simulink model "two_RC_model"  (R2024b)
settings: Solver=VariableStepAuto  StartTime=0.0  StopTime=5000  RelTol=1e-3
undefined symbols (not defined in the file or in its folder): sigbuilder_block
settings Model: Creator=Administrator  LastModifiedBy=sk3547969879
settings DebuggingCC: UnconnectedInputMsg=warning  UnconnectedOutputMsg=warning  UnconnectedLineMsg=warning
settings ModelReferenceCC: EnableRefExpFcnMdlSchedulingChecks=on
settings RTWCC: GPUComputeCapability=3.5  DLArmComputeVersion=19.05

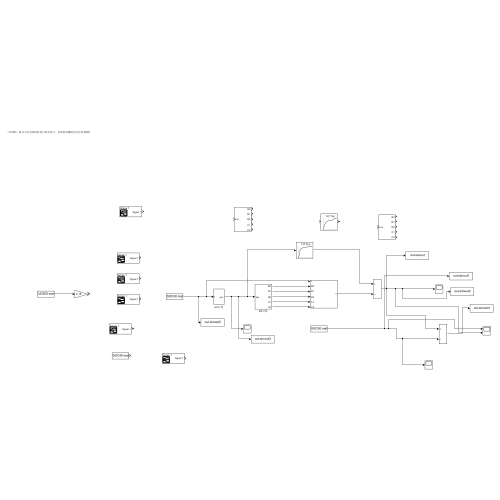
[thumbnail: Simulink's stored preview of the top-level diagram]
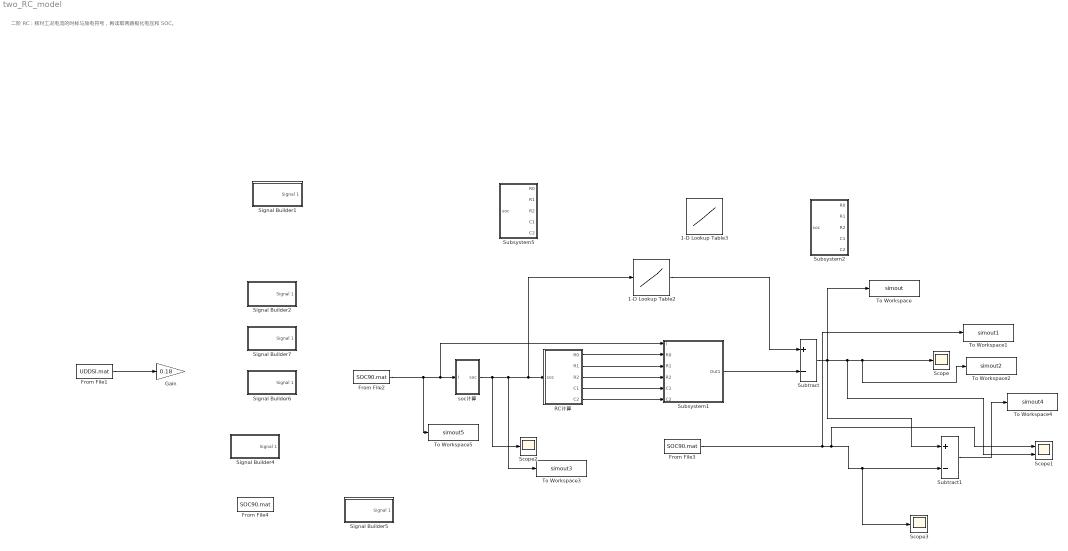
== system two_RC_model ==
  note: 二阶 RC：核对工况电流的时标与放电符号，再读取两路极化电压和 SOC。
  1-D Lookup Table2 : Lookup_n-D  NumberOfTableDimensions=1  BreakpointsForDimension1=[0 0.1 0.2 0.3 0.4 0.5 0.6 0.7 0.8 0.9]  Table=|  InternalRulePriority=Speed  RndMeth=Simplest
      | [2.73200000000000
      | 3.16400000000000
      | 3.21900000000000
      | 3.26100000000000
      | 3.28700000000000
      | 3.28800000000000
      | 3.29100000000000
      | 3.32800000000000
      | 3.32800000000000
      | 3.32900000000000]
  1-D Lookup Table3 : Lookup_n-D  NumberOfTableDimensions=1  BreakpointsForDimension1=[0.1 0.2 0.3 0.4 0.5 0.6 0.7 0.8 0.9]  Table=|  InternalRulePriority=Speed  RndMeth=Simplest
      | [12.8525
      | 13.1367
      | 13.3425
      | 13.3736
      | 13.39
      | 13.4033
      | 13.4506
      | 13.5189
      | 13.5482
      | ]
  From File1 : FromFile  FileName=UDDSI.mat  SampleTime=0
  From File2 : FromFile  FileName=SOC90.mat  SampleTime=0
  From File3 : FromFile  FileName=SOC90.mat  SampleTime=0
  From File4 : FromFile  FileName=SOC90.mat  SampleTime=0
  Gain : Gain  Gain=0.18
  RC计算 : Subsystem
  Scope : Scope
  Scope1 : Scope  NumInputPorts=2
  Scope2 : Scope
  Scope3 : Scope
  Signal Builder1 : Subsystem  Tag=STV Subsys  LoadFcn=sigbuilder_block('load');  StartFcn=sigbuilder_block('start');  StopFcn=sigbuilder_block('stop');  ClipboardFcn=sigbuilder_block('clipboard');  mask(Sigbuilder block){tuvar=[0:10]}
      mask help: Simulink:masks:SigbuilderBlock_MD
      mask init:
      | if ~strcmp(get_param(bdroot(gcbh),'SimulationStatus'),'stopped') tuvar = sigbuilder_block('maskInit'); end
      settings: CopyFcn=sigbuilder_block('copy');  DeleteFcn=sigbuilder_block('delete');  ModelCloseFcn=sigbuilder_block('modelClose');  PreSaveFcn=sigbuilder_block('preSave');  PauseFcn=sigbuilder_block('pause');  ContinueFcn=sigbuilder_block('continue');  NameChangeFcn=sigbuilder_block('namechange');  OpenFcn=sigbuilder_block('open',[437.6 199.2 550.4 400 ]);  CloseFcn=sigbuilder_block('close');
      mask Display: plot(0, 0, 100, 100,[2, 2, 32, 32, 2], [68, 8, 8, 68, 68],[32, 2], [38, 38], [32, 19, 2],[53, 60, 44], [32, 17, 17, 2],[16, 16, 31, 31]);txt = getActiveGroup(gcbh);text(2, 100, txt,'verticalAlignment', 'top');
  Signal Builder2 : Subsystem  Tag=STV Subsys  LoadFcn=sigbuilder_block('load');  StartFcn=sigbuilder_block('start');  StopFcn=sigbuilder_block('stop');  ClipboardFcn=sigbuilder_block('clipboard');  mask(Sigbuilder block){tuvar=[0:10]}
      mask help: Simulink:masks:SigbuilderBlock_MD
      mask init:
      | if ~strcmp(get_param(bdroot(gcbh),'SimulationStatus'),'stopped') tuvar = sigbuilder_block('maskInit'); end
      settings: CopyFcn=sigbuilder_block('copy');  DeleteFcn=sigbuilder_block('delete');  ModelCloseFcn=sigbuilder_block('modelClose');  PreSaveFcn=sigbuilder_block('preSave');  PauseFcn=sigbuilder_block('pause');  ContinueFcn=sigbuilder_block('continue');  NameChangeFcn=sigbuilder_block('namechange');  OpenFcn=sigbuilder_block('open',[437.6 199.2 550.4 400 ]);  CloseFcn=sigbuilder_block('close');
      mask Display: plot(0, 0, 100, 100,[2, 2, 32, 32, 2], [68, 8, 8, 68, 68],[32, 2], [38, 38], [32, 19, 2],[53, 60, 44], [32, 17, 17, 2],[16, 16, 31, 31]);txt = getActiveGroup(gcbh);text(2, 100, txt,'verticalAlignment', 'top');
  Signal Builder4 : Subsystem  Tag=STV Subsys  LoadFcn=sigbuilder_block('load');  StartFcn=sigbuilder_block('start');  StopFcn=sigbuilder_block('stop');  ClipboardFcn=sigbuilder_block('clipboard');  mask(Sigbuilder block){tuvar=[0:10]}
      mask help: Simulink:masks:SigbuilderBlock_MD
      mask init:
      | if ~strcmp(get_param(bdroot(gcbh),'SimulationStatus'),'stopped') tuvar = sigbuilder_block('maskInit'); end
      settings: CopyFcn=sigbuilder_block('copy');  DeleteFcn=sigbuilder_block('delete');  ModelCloseFcn=sigbuilder_block('modelClose');  PreSaveFcn=sigbuilder_block('preSave');  PauseFcn=sigbuilder_block('pause');  ContinueFcn=sigbuilder_block('continue');  NameChangeFcn=sigbuilder_block('namechange');  OpenFcn=sigbuilder_block('open',[6 36 1428 674.25 ]);  CloseFcn=sigbuilder_block('close');
      mask Display: plot(0, 0, 100, 100,[2, 2, 32, 32, 2], [68, 8, 8, 68, 68],[32, 2], [38, 38], [32, 19, 2],[53, 60, 44], [32, 17, 17, 2],[16, 16, 31, 31]);txt = getActiveGroup(gcbh);text(2, 100, txt,'verticalAlignment', 'top');
  Signal Builder5 : Subsystem  Tag=STV Subsys  LoadFcn=sigbuilder_block('load');  StartFcn=sigbuilder_block('start');  StopFcn=sigbuilder_block('stop');  ClipboardFcn=sigbuilder_block('clipboard');  mask(Sigbuilder block){tuvar=[0:10]}
      mask help: Simulink:masks:SigbuilderBlock_MD
      mask init:
      | if ~strcmp(get_param(bdroot(gcbh),'SimulationStatus'),'stopped') tuvar = sigbuilder_block('maskInit'); end
      settings: CopyFcn=sigbuilder_block('copy');  DeleteFcn=sigbuilder_block('delete');  ModelCloseFcn=sigbuilder_block('modelClose');  PreSaveFcn=sigbuilder_block('preSave');  PauseFcn=sigbuilder_block('pause');  ContinueFcn=sigbuilder_block('continue');  NameChangeFcn=sigbuilder_block('namechange');  OpenFcn=sigbuilder_block('open',[437.6 199.2 550.4 400 ]);  CloseFcn=sigbuilder_block('close');
      mask Display: plot(0, 0, 100, 100,[2, 2, 32, 32, 2], [68, 8, 8, 68, 68],[32, 2], [38, 38], [32, 19, 2],[53, 60, 44], [32, 17, 17, 2],[16, 16, 31, 31]);txt = getActiveGroup(gcbh);text(2, 100, txt,'verticalAlignment', 'top');
  Signal Builder6 : Subsystem  Tag=STV Subsys  LoadFcn=sigbuilder_block('load');  StartFcn=sigbuilder_block('start');  StopFcn=sigbuilder_block('stop');  ClipboardFcn=sigbuilder_block('clipboard');  mask(Sigbuilder block){tuvar=[0:10]}
      mask help: Simulink:masks:SigbuilderBlock_MD
      mask init:
      | if ~strcmp(get_param(bdroot(gcbh),'SimulationStatus'),'stopped') tuvar = sigbuilder_block('maskInit'); end
      settings: CopyFcn=sigbuilder_block('copy');  DeleteFcn=sigbuilder_block('delete');  ModelCloseFcn=sigbuilder_block('modelClose');  PreSaveFcn=sigbuilder_block('preSave');  PauseFcn=sigbuilder_block('pause');  ContinueFcn=sigbuilder_block('continue');  NameChangeFcn=sigbuilder_block('namechange');  OpenFcn=sigbuilder_block('open',[437.6 199.2 550.4 400 ]);  CloseFcn=sigbuilder_block('close');
      mask Display: plot(0, 0, 100, 100,[2, 2, 32, 32, 2], [68, 8, 8, 68, 68],[32, 2], [38, 38], [32, 19, 2],[53, 60, 44], [32, 17, 17, 2],[16, 16, 31, 31]);txt = getActiveGroup(gcbh);text(2, 100, txt,'verticalAlignment', 'top');
  Signal Builder7 : Subsystem  Tag=STV Subsys  LoadFcn=sigbuilder_block('load');  StartFcn=sigbuilder_block('start');  StopFcn=sigbuilder_block('stop');  ClipboardFcn=sigbuilder_block('clipboard');  mask(Sigbuilder block){tuvar=[0:10]}
      mask help: Simulink:masks:SigbuilderBlock_MD
      mask init:
      | if ~strcmp(get_param(bdroot(gcbh),'SimulationStatus'),'stopped') tuvar = sigbuilder_block('maskInit'); end
      settings: CopyFcn=sigbuilder_block('copy');  DeleteFcn=sigbuilder_block('delete');  ModelCloseFcn=sigbuilder_block('modelClose');  PreSaveFcn=sigbuilder_block('preSave');  PauseFcn=sigbuilder_block('pause');  ContinueFcn=sigbuilder_block('continue');  NameChangeFcn=sigbuilder_block('namechange');  OpenFcn=sigbuilder_block('open',[4.875 36 1190.25 638.25 ]);  CloseFcn=sigbuilder_block('close');
      mask Display: plot(0, 0, 100, 100,[2, 2, 32, 32, 2], [68, 8, 8, 68, 68],[32, 2], [38, 38], [32, 19, 2],[53, 60, 44], [32, 17, 17, 2],[16, 16, 31, 31]);txt = getActiveGroup(gcbh);text(2, 100, txt,'verticalAlignment', 'top');
  Subsystem1 : Subsystem
  Subsystem2 : Subsystem
  Subsystem5 : Subsystem
  Subtract : Sum  Inputs=+-
  Subtract1 : Sum  Inputs=+-
  To Workspace : ToWorkspace  VariableName=simout  SampleTime=1
  To Workspace1 : ToWorkspace  VariableName=simout1  SampleTime=1
  To Workspace2 : ToWorkspace  VariableName=simout2  SampleTime=1
  To Workspace3 : ToWorkspace  VariableName=simout3  SampleTime=1
  To Workspace4 : ToWorkspace  VariableName=simout4  SampleTime=1
  To Workspace5 : ToWorkspace  VariableName=simout5  SampleTime=1
  soc计算 : Subsystem
  wires:
  Subtract1/1 -> To Workspace4/1
  RC计算/2(R1) -> Subsystem1/3(R1)
  From File3/1 -> To Workspace1/1, Scope1/1, Scope3/1, Subtract1/2
  RC计算/4(C1) -> Subsystem1/5(C1)
  From File1/1 -> Gain/1
  RC计算/3(R2) -> Subsystem1/4(R2)
  Subtract/1 -> To Workspace/1, Scope1/2, To Workspace2/1, Scope/1, Subtract1/1
  soc计算/1(soc) -> Scope2/1, To Workspace3/1, RC计算/1(soc), 1-D Lookup Table2/1
  RC计算/1(R0) -> Subsystem1/2(R0)
  1-D Lookup Table2/1 -> Subtract/1
  Subsystem1/1(Out1) -> Subtract/2
  RC计算/5(C2) -> Subsystem1/6(C2)
  From File2/1 -> To Workspace5/1, Subsystem1/1(I), soc计算/1(I)

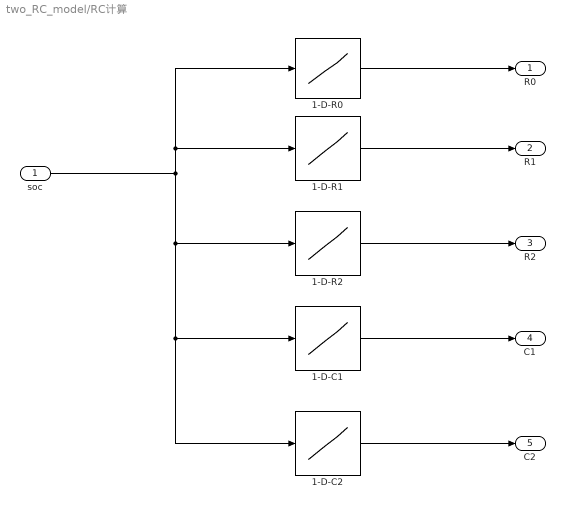
== system two_RC_model/RC计算 ==
  soc : Inport
  1-D-C1 : Lookup_n-D  NumberOfTableDimensions=1  BreakpointsForDimension1=[0.1 0.9]  Table=[230209.202612874 230209.202612874]  InternalRulePriority=Speed  RndMeth=Simplest
  1-D-C2 : Lookup_n-D  NumberOfTableDimensions=1  BreakpointsForDimension1=[0.1 0.9]  Table=[1155798.78698917 1155798.78698917]  InternalRulePriority=Speed  RndMeth=Simplest
  1-D-R0 : Lookup_n-D  NumberOfTableDimensions=1  BreakpointsForDimension1=[0.1 0.9]  Table=[0.0011 0.0011]  InternalRulePriority=Speed  RndMeth=Simplest
  1-D-R1 : Lookup_n-D  NumberOfTableDimensions=1  BreakpointsForDimension1=[0.1 0.9]  Table=[0.000589 0.000589]  InternalRulePriority=Speed  RndMeth=Simplest
  1-D-R2 : Lookup_n-D  NumberOfTableDimensions=1  BreakpointsForDimension1=[0.1 0.9]  Table=[0.0009175 0.0009175]  InternalRulePriority=Speed  RndMeth=Simplest
  R0 : Outport
  R1 : Outport  Port=2
  R2 : Outport  Port=3
  C1 : Outport  Port=4
  C2 : Outport  Port=5
  wires:
  1-D-R2/1 -> R2/1
  soc/1 -> 1-D-C2/1, 1-D-C1/1, 1-D-R2/1, 1-D-R1/1, 1-D-R0/1
  1-D-R1/1 -> R1/1
  1-D-C1/1 -> C1/1
  1-D-C2/1 -> C2/1
  1-D-R0/1 -> R0/1

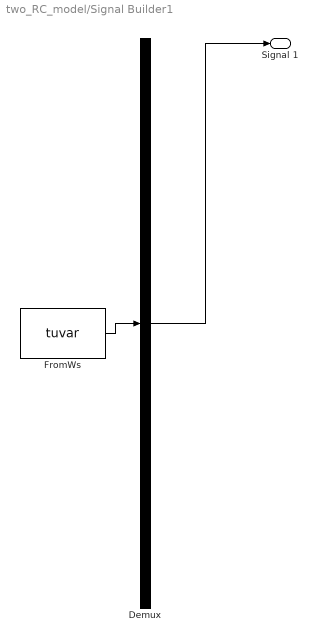
== system two_RC_model/Signal Builder1 ==
  Demux : Demux  Tag=STV Demux  Outputs=1
      settings: DisplayOption=none
  FromWs : FromWorkspace  Tag=STV FromWs  VariableName=tuvar
      SigBuilderData=|
      | common.afterFinalStr = 'Extrapolate'
      | common.sampleTime = 0
      | dataSet.timeRange = [0 7000]
      | dataSet.name = 'Group 1'
      | sbobj.Groups.Name = 'Group 1'
      | sbobj.Groups.Signals.Name = 'Signal 1'
      | sbobj.Groups.Signals.XData = [0 1800 1800 2523 2523 6124 6124 6845 6845 7000]
      | sbobj.Groups.Signals.YData = [0 0 20 20 0 0 20 20 0 0]
      | sbobj.Groups.TimeRange = [0 7000]
  Signal 1 : Outport  Tag=STV Outport
  wires:
  FromWs/1 -> Demux/1
  Demux/1 -> Signal 1/1

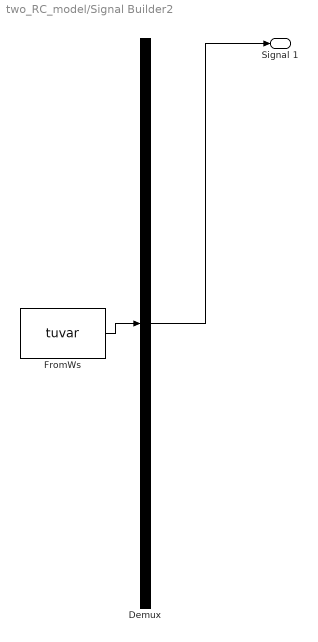
== system two_RC_model/Signal Builder2 ==
  Demux : Demux  Tag=STV Demux  Outputs=1
      settings: DisplayOption=none
  FromWs : FromWorkspace  Tag=STV FromWs  VariableName=tuvar
      SigBuilderData=|
      | common.afterFinalStr = 'Extrapolate'
      | common.sampleTime = 0
      | dataSet.timeRange = [0 7000]
      | dataSet.name = 'Group 1'
      | sbobj.Groups.Name = 'Group 1'
      | sbobj.Groups.Signals.Name = 'Signal 1'
      | sbobj.Groups.Signals.XData = [0 1800 1800 2523 2523 6124 6124 6845 6845 7000]
      | sbobj.Groups.Signals.YData = [0 0 20 20 0 0 20 20 0 0]
      | sbobj.Groups.TimeRange = [0 7000]
  Signal 1 : Outport  Tag=STV Outport
  wires:
  Demux/1 -> Signal 1/1
  FromWs/1 -> Demux/1

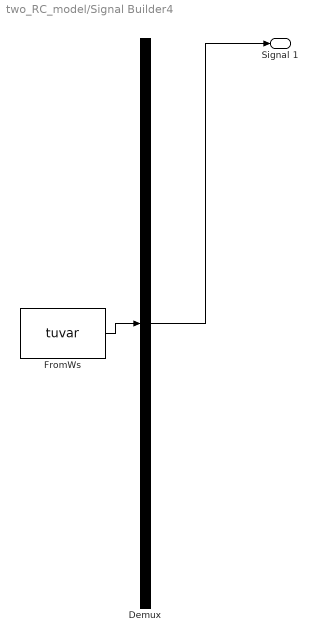
== system two_RC_model/Signal Builder4 ==
  Demux : Demux  Tag=STV Demux  Outputs=1
      settings: DisplayOption=none
  FromWs : FromWorkspace  Tag=STV FromWs  VariableName=tuvar
      SigBuilderData=|
      | common.afterFinalStr = 'Extrapolate'
      | common.sampleTime = 0
      | dataSet.timeRange = [0 10000]
      | dataSet.name = 'Group 1'
      | sbobj.Groups.Name = 'Group 1'
      | sbobj.Groups.Signals.Name = 'Signal 1'
      | sbobj.Groups.Signals.XData = [0 240 240 1160 1160 1820 1820 2840 2840 3660 3660 4750 4750 5720 5720 6650 6650 7340 7340 8300 8300 9070 9070 9840 9840 10000]
      | sbobj.Groups.Signals.YData = [0 0 21.15 21.15 4.1 4.1 16.15 16.15 -2.2 -2.2 22 22 0 0 19.95 19.95 -1.2 -1.2 19.95 19.95 1.45 1.45 19.9 19.9 0 0]
      | sbobj.Groups.TimeRange = [0 10000]
  Signal 1 : Outport  Tag=STV Outport
  wires:
  Demux/1 -> Signal 1/1
  FromWs/1 -> Demux/1

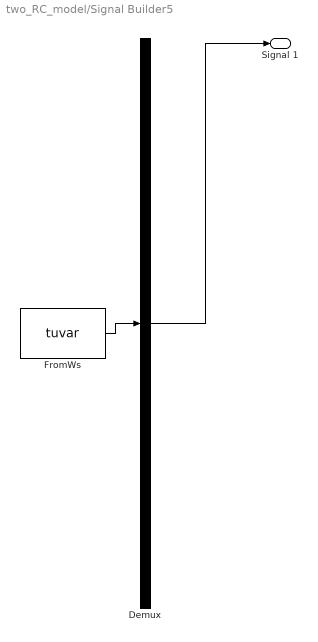
== system two_RC_model/Signal Builder5 ==
  Demux : Demux  Tag=STV Demux  Outputs=1
      settings: DisplayOption=none
  FromWs : FromWorkspace  Tag=STV FromWs  VariableName=tuvar
      SigBuilderData=|
      | common.afterFinalStr = 'Extrapolate'
      | common.sampleTime = 0
      | dataSet.timeRange = [0 7000]
      | dataSet.name = 'Group 1'
      | sbobj.Groups.Name = 'Group 1'
      | sbobj.Groups.Signals.Name = 'Signal 1'
      | sbobj.Groups.Signals.XData = [0 500 500 1260 1260 1960 1960 2800 2800 3520 3520 4220 4220 4940 4940 5660 5660 6380 6380 6900 6900 7000]
      | sbobj.Groups.Signals.YData = [0 0 20 20 0 0 20 20 0 0 19.9 19.9 0 0 19.9 19.9 0 0 19.9 19.9 0 0]
      | sbobj.Groups.TimeRange = [0 7000]
  Signal 1 : Outport  Tag=STV Outport
  wires:
  Demux/1 -> Signal 1/1
  FromWs/1 -> Demux/1

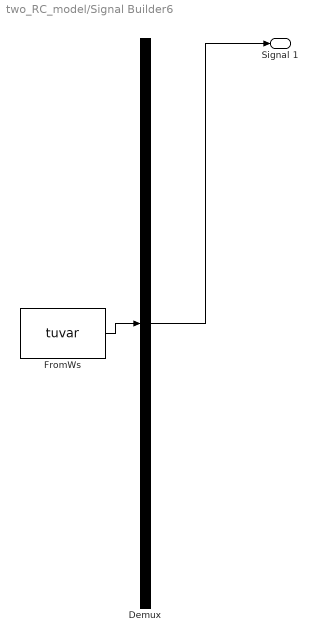
== system two_RC_model/Signal Builder6 ==
  Demux : Demux  Tag=STV Demux  Outputs=1
      settings: DisplayOption=none
  FromWs : FromWorkspace  Tag=STV FromWs  VariableName=tuvar
      SigBuilderData=|
      | common.afterFinalStr = 'Extrapolate'
      | common.sampleTime = 0
      | dataSet.timeRange = [0 7000]
      | dataSet.name = 'Group 1'
      | sbobj.Groups.Name = 'Group 1'
      | sbobj.Groups.Signals.Name = 'Signal 1'
      | sbobj.Groups.Signals.XData = [0 1800 1800 2523 2523 6124 6124 6845 6845 7000]
      | sbobj.Groups.Signals.YData = [0 0 20 20 0 0 20 20 0 0]
      | sbobj.Groups.TimeRange = [0 7000]
  Signal 1 : Outport  Tag=STV Outport
  wires:
  Demux/1 -> Signal 1/1
  FromWs/1 -> Demux/1

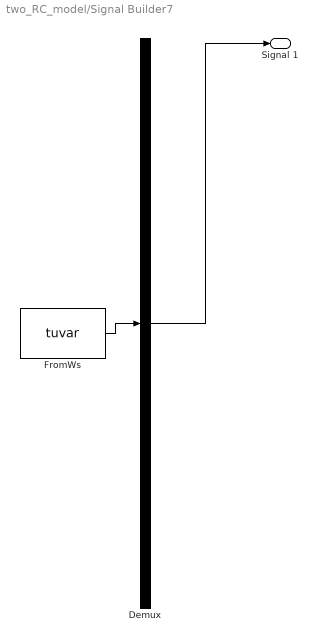
== system two_RC_model/Signal Builder7 ==
  Demux : Demux  Tag=STV Demux  Outputs=1
      settings: DisplayOption=none
  FromWs : FromWorkspace  Tag=STV FromWs  VariableName=tuvar
      SigBuilderData=|
      | common.afterFinalStr = 'Extrapolate'
      | common.sampleTime = 0
      | dataSet.timeRange = [0 10000]
      | dataSet.name = 'Group 1'
      | sbobj.Groups.Name = 'Group 1'
      | sbobj.Groups.Signals.Name = 'Signal 1'
      | sbobj.Groups.Signals.XData = [0 240 1800 1800 2550 2550 3660 4750 5720 6650 7340 8300 9070 9840 10000]
      | sbobj.Groups.Signals.YData = [0 0 0 20 20 0 0 0 0 0 0 0 0 0 0]
      | sbobj.Groups.TimeRange = [0 10000]
  Signal 1 : Outport  Tag=STV Outport
  wires:
  Demux/1 -> Signal 1/1
  FromWs/1 -> Demux/1

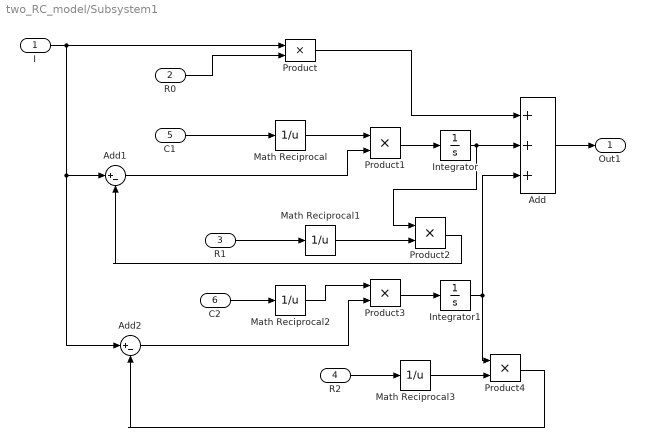
== system two_RC_model/Subsystem1 ==
  I : Inport
  R0 : Inport  Port=2
  R1 : Inport  Port=3
  R2 : Inport  Port=4
  C1 : Inport  Port=5
  C2 : Inport  Port=6
  Add : Sum  Inputs=+++
  Add1 : Sum  Inputs=|+-
  Add2 : Sum  Inputs=|+-
  Integrator : Integrator
  Integrator1 : Integrator
  Math Reciprocal{,1..3} (4 alike) : Math  Operator=reciprocal  SignedPower=on
  Product{,1..4} (5 alike) : Product
  Out1 : Outport
  wires:
  Math Reciprocal1/1 -> Product2/2
  R1/1 -> Math Reciprocal1/1
  Product2/1 -> Add1/2
  R2/1 -> Math Reciprocal3/1
  Math Reciprocal3/1 -> Product4/2
  R0/1 -> Product/2
  C1/1 -> Math Reciprocal/1
  I/1 -> Add2/1, Add1/1, Product/1
  C2/1 -> Math Reciprocal2/1
  Product4/1 -> Add2/2
  Product/1 -> Add/1
  Math Reciprocal/1 -> Product1/1
  Add1/1 -> Product1/2
  Math Reciprocal2/1 -> Product3/1
  Add2/1 -> Product3/2
  Product1/1 -> Integrator/1
  Product3/1 -> Integrator1/1
  Integrator/1 -> Product2/1, Add/2
  Integrator1/1 -> Product4/1, Add/3
  Add/1 -> Out1/1

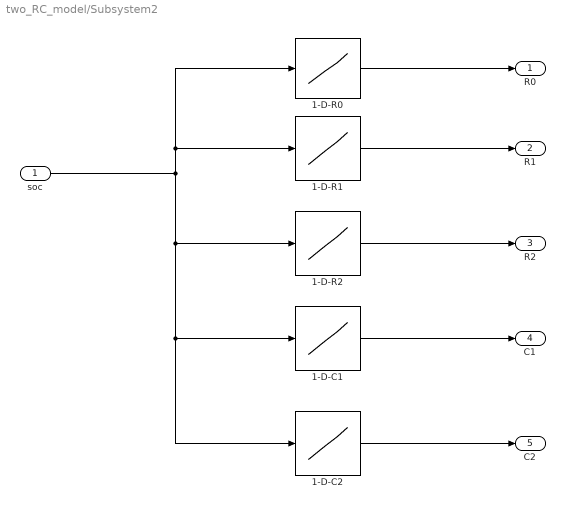
== system two_RC_model/Subsystem2 ==
  soc : Inport
  1-D-C1 : Lookup_n-D  NumberOfTableDimensions=1  BreakpointsForDimension1=[0.1 0.9]  Table=[5000 5000]  InternalRulePriority=Speed  RndMeth=Simplest
  1-D-C2 : Lookup_n-D  NumberOfTableDimensions=1  BreakpointsForDimension1=[0.1 0.9]  Table=[1200 1200]  InternalRulePriority=Speed  RndMeth=Simplest
  1-D-R0 : Lookup_n-D  NumberOfTableDimensions=1  BreakpointsForDimension1=[0.1 0.9]  Table=[0.05 0.05]  InternalRulePriority=Speed  RndMeth=Simplest
  1-D-R1 : Lookup_n-D  NumberOfTableDimensions=1  BreakpointsForDimension1=[0.1 0.9]  Table=[0.2638 0.2638]  InternalRulePriority=Speed  RndMeth=Simplest
  1-D-R2 : Lookup_n-D  NumberOfTableDimensions=1  BreakpointsForDimension1=[0.1 0.9]  Table=[0.00038 0.00038]  InternalRulePriority=Speed  RndMeth=Simplest
  R0 : Outport
  R1 : Outport  Port=2
  R2 : Outport  Port=3
  C1 : Outport  Port=4
  C2 : Outport  Port=5
  wires:
  1-D-R2/1 -> R2/1
  soc/1 -> 1-D-C2/1, 1-D-C1/1, 1-D-R2/1, 1-D-R1/1, 1-D-R0/1
  1-D-R1/1 -> R1/1
  1-D-C1/1 -> C1/1
  1-D-C2/1 -> C2/1
  1-D-R0/1 -> R0/1

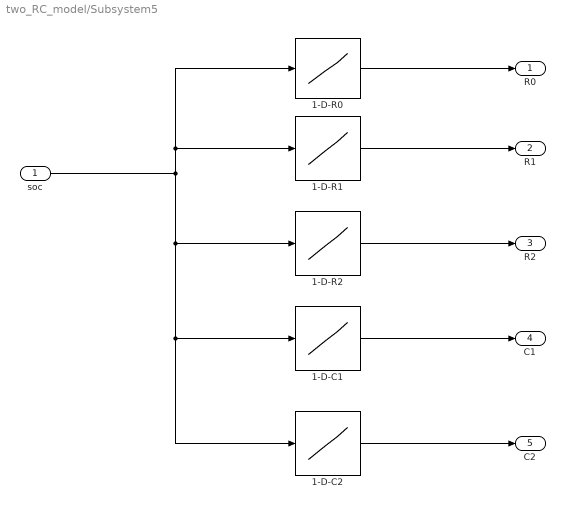
== system two_RC_model/Subsystem5 ==
  soc : Inport
  1-D-C1 : Lookup_n-D  NumberOfTableDimensions=1  BreakpointsForDimension1=[0 0.1 0.2 0.3 0.4 0.5 0.6 0.7 0.8 0.9]  Table=|  InternalRulePriority=Speed  RndMeth=Simplest
      | [2.21E+03	5.69E+04	2.54E+04	1.69E+05	1.22E+05	1.97E+05	1.83E+05	8.64E+04	2.27E+05	2.30E+05
      | 
      | ]
  1-D-C2 : Lookup_n-D  NumberOfTableDimensions=1  BreakpointsForDimension1=[0 0.1 0.2 0.3 0.4 0.5 0.6 0.7 0.8 0.9]  Table=|  InternalRulePriority=Speed  RndMeth=Simplest
      | [1.68E+06	1.75E+06	8.40E+07	1.45E+06	1.44E+06	1.61E+06	1.81E+06	2.92E+06	2.39E+06	1.16E+06
      | ]
  1-D-R0 : Lookup_n-D  NumberOfTableDimensions=1  BreakpointsForDimension1=[0 0.1 0.2 0.3 0.4 0.5 0.6 0.7 0.8 0.9]  Table=|  InternalRulePriority=Speed  RndMeth=Simplest
      | [0.0025	0.0019	0.00145	0.0013	0.00145	0.00125	0.00115	0.0014	0.00125	0.0011
      | ]
  1-D-R1 : Lookup_n-D  NumberOfTableDimensions=1  BreakpointsForDimension1=[0 0.1 0.2 0.3 0.4 0.5 0.6 0.7 0.8 0.9]  Table=|  InternalRulePriority=Speed  RndMeth=Simplest
      | [3.76E-03	0.001134	8.09E-04	5.61E-04	6.64E-04	5.18E-04	5.96E-04	7.99E-04	5.56E-04	5.89E-04
      | ]
  1-D-R2 : Lookup_n-D  NumberOfTableDimensions=1  BreakpointsForDimension1=[0 0.1 0.2 0.3 0.4 0.5 0.6 0.7 0.8 0.9]  Table=|  InternalRulePriority=Speed  RndMeth=Simplest
      | [5.95E-04	5.69E-04	2.66E-04	6.48E-04	6.05E-04	6.40E-04	6.51E-04	3.52E-04	5.94E-04	9.18E-04
      | ]
  R0 : Outport
  R1 : Outport  Port=2
  R2 : Outport  Port=3
  C1 : Outport  Port=4
  C2 : Outport  Port=5
  wires:
  1-D-R0/1 -> R0/1
  1-D-C2/1 -> C2/1
  1-D-C1/1 -> C1/1
  1-D-R1/1 -> R1/1
  soc/1 -> 1-D-R0/1, 1-D-R1/1, 1-D-R2/1, 1-D-C1/1, 1-D-C2/1
  1-D-R2/1 -> R2/1

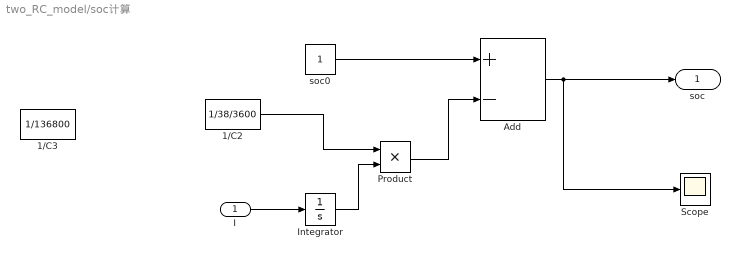
== system two_RC_model/soc计算 ==
  I : Inport
  1/C2 : Constant  Value=1/38/3600
  1/C3 : Constant  Value=1/136800
  Add : Sum  Inputs=+-
  Integrator : Integrator
  Product : Product
  Scope : Scope
  soc0 : Constant
  soc : Outport
  wires:
  1/C2/1 -> Product/1
  soc0/1 -> Add/1
  Add/1 -> soc/1, Scope/1
  Product/1 -> Add/2
  Integrator/1 -> Product/2
  I/1 -> Integrator/1
